simulink model "sf_data_event_msg"  (R2025b)
settings: Solver=FixedStepDiscrete  StartTime=0.0  StopTime=10.0  FixedStep=1  RelTol=1e-3  EnableMultiTasking=on
settings Model: Creator=The MathWorks, Inc.  LastModifiedBy=The MathWorks, Inc.
settings SolverCC: AlgebraicLoopSolver=TrustRegion
settings DataIOCC: LimitDataPoints=on  SaveFormat=Array  ReturnWorkspaceOutputs=off
settings OptimizationCC: ReuseModelBlockBuffer=off  ExpressionDepthLimit=2147483647.0  LifeSpan=1  EfficientTunableParamExpr=on
settings DebuggingCC: UnderspecifiedInitializationDetection=Classic  MergeDetectMultiDrivingBlocksExec=none  SolverPrmCheckMsg=warning  UnconnectedInputMsg=warning  UnconnectedOutputMsg=warning  UnconnectedLineMsg=warning  AllowSymbolicDim=off  StateNameClashWarn=warning  SFUnexpectedBacktrackingDiag=warning  SFNoUnconditionalDefaultTransitionDiag=warning  SFExecutionAtInitializationDiag=none  ArithmeticOperatorsInVariantConditions=warning
settings HardwareCC: ProdBitPerPointer=32.0  ProdBitPerSizeT=32.0  ProdBitPerPtrDiffT=32.0  ProdLargestAtomicFloat=None  ProdIntDivRoundTo=Undefined  ProdEndianess=Unspecified  ProdWordSize=32.0  ProdHWDeviceType=32-bit Generic
settings ModelReferenceCC: EnableRefExpFcnMdlSchedulingChecks=on  PropagateSignalLabelsOutOfModel=off
settings SFSimCC: SimUseLocalCustomCode=off  MATLABDynamicMemAlloc=off
settings RTWCC: SystemTargetFile=ert.tlc  TemplateMakefile=ert_default_tmf  RTWUseLocalCustomCode=off  GPUComputeCapability=3.5  DLArmComputeVersion=19.05  Description=Real-Time Workshop Embedded Coder
settings CodeAppCC: IgnoreCustomStorageClasses=off  CustomSymbolStrType=$N$R$M  StateflowObjectComments=on  InternalIdentifier=Classic
settings ERTTargetCC: InlinedParameterPlacement=Hierarchical  ERTCustomFileTemplate=example_file_process.tlc  ConvertIfToSwitch=off  SuppressUnreachableDefaultCases=off  MultiwordLength=2048.0  GenerateSampleERTMain=on
settings ConfigComp: CovMetricSettings=dw  CovSaveCumulativeToWorkspaceVar=on  CovSaveSingleToWorkspaceVar=on  CovExternalEMLEnable=off  CovSFcnEnable=off

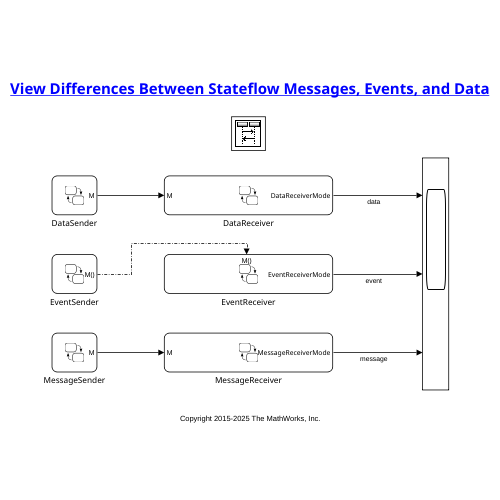
[thumbnail: Simulink's stored preview of the top-level diagram]
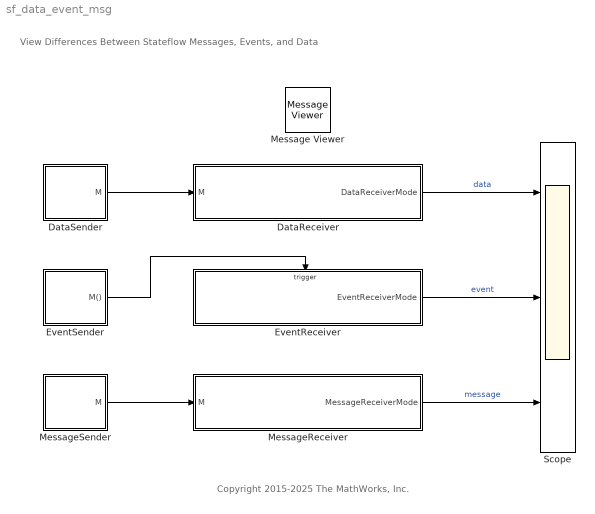
== system sf_data_event_msg ==
  note: Copyright 2015-2025 The MathWorks, Inc.
  note: View Differences Between Stateflow Messages, Events, and Data
  DataReceiver : Stateflow chart  TreatAsAtomicUnit=on
  DataSender : Stateflow chart  TreatAsAtomicUnit=on
  EventReceiver : Stateflow chart  TreatAsAtomicUnit=on
  EventSender : Stateflow chart  TreatAsAtomicUnit=on
  Message Viewer : MessageViewer  SavedRootId=#
  MessageReceiver : Stateflow chart  TreatAsAtomicUnit=on
  MessageSender : Stateflow chart  TreatAsAtomicUnit=on
  Scope : Scope  NumInputPorts=3
      settings: ActiveDisplayYMinimum=0  ActiveDisplayYMaximum=5
  wires:
  MessageSender/1(M) -> MessageReceiver/1(M)
  EventSender/1(M()) -> EventReceiver/Trigger
  DataSender/1(M) -> DataReceiver/1(M)
  EventReceiver/1(EventReceiverMode) -> Scope/2  "event"
  MessageReceiver/1(MessageReceiverMode) -> Scope/3  "message"
  DataReceiver/1(DataReceiverMode) -> Scope/1  "data"

== stateflow chart sf_data_event_msg/MessageSender ==
  state A
    en:
    send(M);
  (default) -> A
  data: M output double

== stateflow chart sf_data_event_msg/MessageReceiver ==
  state A0
  state A1
  state A2
  state A3
  (default) -> A0
  A0 -> A1 : after(3,sec)
  A1 -> A2 : M
  A2 -> A3 : M
  data: M input double; MessageReceiverMode output Enum: MessageReceiverModeType

== stateflow chart sf_data_event_msg/EventReceiver ==
  state A0
  state A1
  state A2
  state A3
  (default) -> A0
  A0 -> A1 : after(3,sec)
  A1 -> A2 : M
  A2 -> A3 : M
  data: EventReceiverMode output Enum: EventReceiverModeType
  events: M input FUNCTION_CALL_EVENT

== stateflow chart sf_data_event_msg/EventSender ==
  state A
    en:
    send(M)
  (default) -> A
  events: M output FUNCTION_CALL_EVENT

== stateflow chart sf_data_event_msg/DataReceiver ==
  state A0
  state A1
  state A2
  state A3
  (default) -> A0
  A0 -> A1 : after(3,sec)
  A1 -> A2 : [M == 1]
  A2 -> A3 : [M == 1]
  data: M input double; DataReceiverMode output Enum: DataReceiverModeType

== stateflow chart sf_data_event_msg/DataSender ==
  state A
    en:
    M = 1;
  (default) -> A
  data: M output double
